simulink subsystem "DCMInclinedOrbitLN"  (R2024b)
settings: Solver=VariableStepAuto  StartTime=0.0  StopTime=10.0  RelTol=1e-3
settings Model: Creator=marco  LastModifiedBy=ferru

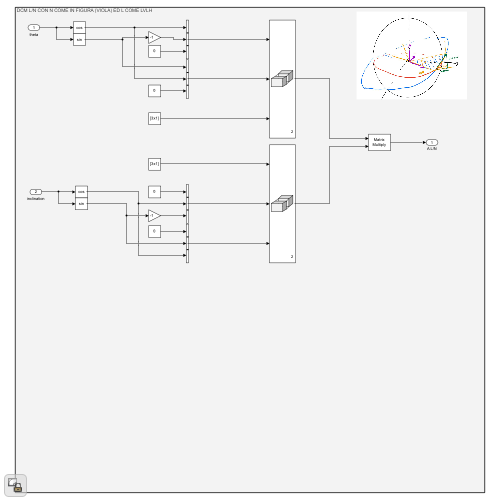
[thumbnail: Simulink's stored preview of the top-level diagram]
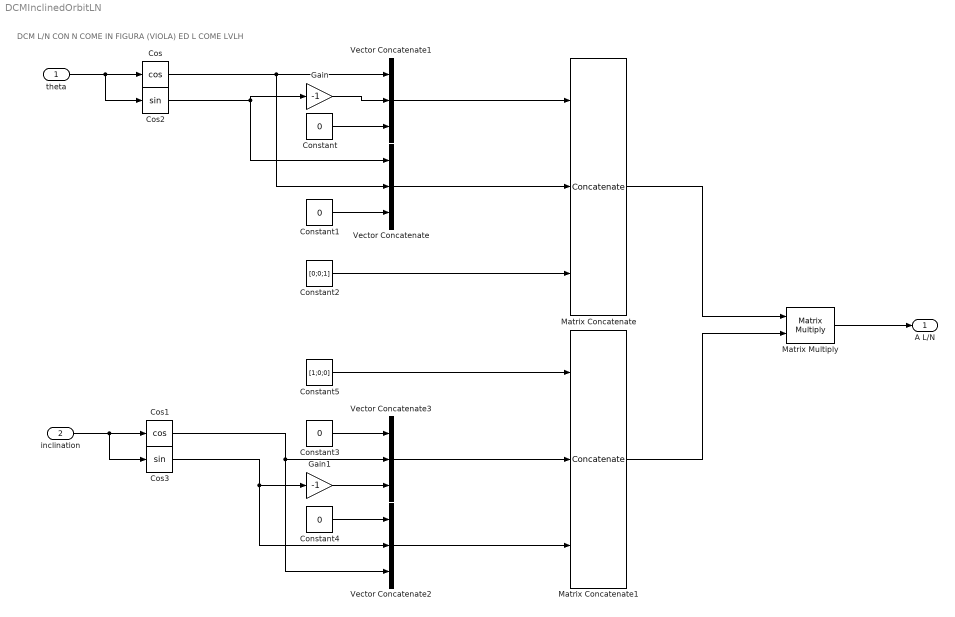
== system DCMInclinedOrbitLN ==
  note: DCM L/N CON N COME IN FIGURA (VIOLA) ED L COME LVLH
  theta : Inport
  inclination : Inport  Port=2
  Constant{,1,3..4} (4 alike) : Constant  Value=0
  Constant2 : Constant  Value=[0;0;1]
  Constant5 : Constant  Value=[1;0;0]
  Cos : Trigonometry  Operator=cos
  Cos1 : Trigonometry  Operator=cos
  Cos2 : Trigonometry
  Cos3 : Trigonometry
  Gain : Gain  Gain=-1
  Gain1 : Gain  Gain=-1
  Matrix Concatenate : Concatenate  NumInputs=3  Mode=Multidimensional array  ConcatenateDimension=2
  Matrix Concatenate1 : Concatenate  NumInputs=3  Mode=Multidimensional array  ConcatenateDimension=2
  Matrix Multiply : Product  Multiplication=Matrix(*)
  Vector Concatenate{,1..3} (4 alike) : Concatenate  NumInputs=3
  A L/N : Outport
  wires:
  theta/1 -> Cos/1, Cos2/1
  inclination/1 -> Cos1/1, Cos3/1
  Cos/1 -> Vector Concatenate1/1, Vector Concatenate/2
  Cos2/1 -> Gain/1, Vector Concatenate/1
  Gain/1 -> Vector Concatenate1/2
  Constant/1 -> Vector Concatenate1/3
  Constant1/1 -> Vector Concatenate/3
  Vector Concatenate1/1 -> Matrix Concatenate/1
  Vector Concatenate/1 -> Matrix Concatenate/2
  Constant2/1 -> Matrix Concatenate/3
  Constant5/1 -> Matrix Concatenate1/1
  Vector Concatenate2/1 -> Matrix Concatenate1/3
  Vector Concatenate3/1 -> Matrix Concatenate1/2
  Cos3/1 -> Gain1/1, Vector Concatenate2/2
  Cos1/1 -> Vector Concatenate3/2, Vector Concatenate2/3
  Gain1/1 -> Vector Concatenate3/3
  Constant3/1 -> Vector Concatenate3/1
  Constant4/1 -> Vector Concatenate2/1
  Matrix Concatenate/1 -> Matrix Multiply/1
  Matrix Concatenate1/1 -> Matrix Multiply/2
  Matrix Multiply/1 -> A L/N/1
